simulink model "mainEMDmode"  (R2025b)
settings: Solver=VariableStepAuto  StartTime=0.0  StopTime=10  RelTol=1e-3
values from neighbouring files (symbols this model uses):
  B_m = (kfi^2*I_anl)/(V_an-R_a*I_anl)    (= 3.63928112965e-07)    [mainEMD.m]    (also in matlab.mat)
  Denominator = [L_a*J_m* + (L_a*B_m + J_m*R_a) + R_a*B_m+kfi^2]    [mainEMD.m]    (also in matlab.mat = 0.000519897304237)
  J_m = 1.16*10^-7    (= 1.16e-07)    [mainEMD.m]    (also in matlab.mat)
  kfi = 0.0225    [mainEMD.m]    (also in matlab.mat)
  L_a = 0.00137    [mainEMD.m]    (also in matlab.mat)
  Numerator = [kfi]    [mainEMD.m]    (also in matlab.mat = 0.0225)
  R_a = 37.5    [mainEMD.m]    (also in matlab.mat)
  T_n = 4.76*10^-3    (= 0.00476)    [mainEMD.m]    (also in matlab.mat)
  V_an = 24    [mainEMD.m]    (also in matlab.mat)
libraries: fl_lib x6, nesl_utility x5, ee_lib x2
settings Model: Creator=osakwe  LastModifiedBy=osakwe

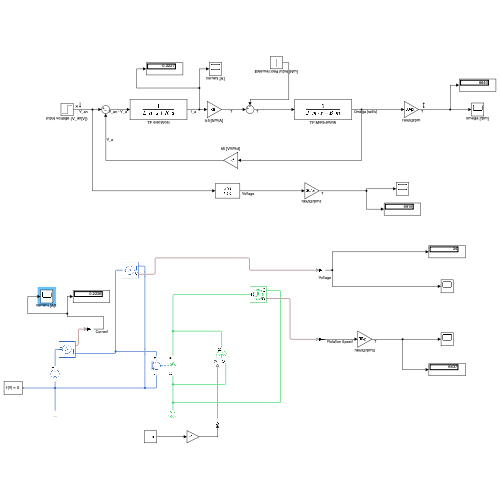
[thumbnail: Simulink's stored preview of the top-level diagram]
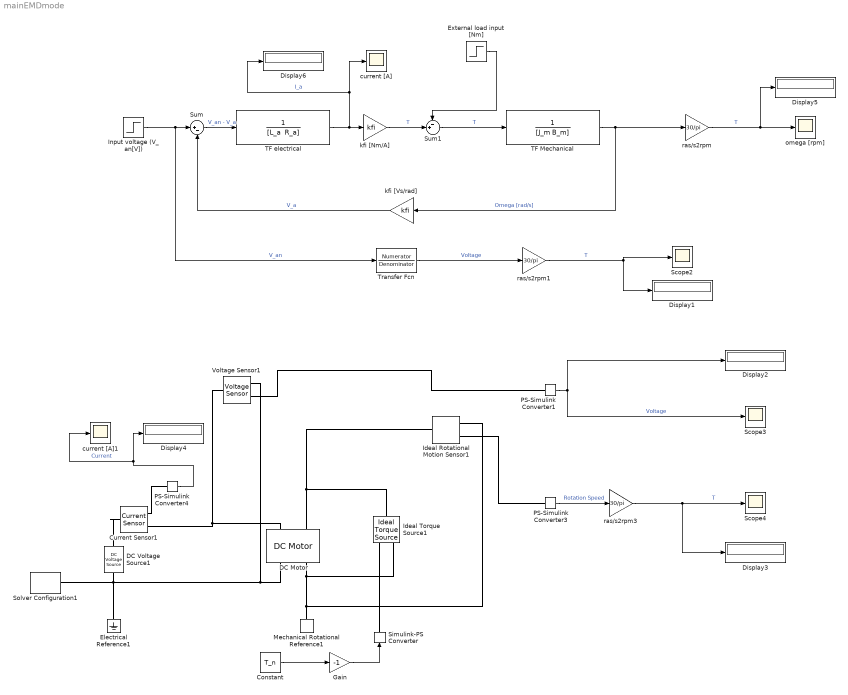
== system mainEMDmode ==
  Constant : Constant  Value=T_n
  Current Sensor1 : fl_lib/Electrical/Electrical Sensors/Current Sensor
  DC Motor : ee_lib/Electromechanical/Brushed Motors/DC Motor  field_option=ee.enum.field_option.pm  Rf=100 Ohm  Lf=1 H  Laf=0.15 H  If0=0 A  parameterization=ee.enum.dcparam_option.circuit_param  Ra=37.5 Ohm  La=1.37 mH  emf_or_torque=ee.enum.emf_or_torque.kv  Kv=0.00235849 V/rpm  Ki=6.876e-4 N*m/A  T_stall=14.4 mN*m  w_max=9920 rpm  w_rated=15000 rpm  P_rated=0.08 W  V_rated=1.5 V  lam_param=ee.enum.lam_param.damping  i_noload=16.8 mA  V_i_noload=1.5 V  J=1.16 cm^2*g  lam=B_m N*m*s/rad  speed0=0 rpm  alpha=3.93e-3 1/K  Tmeas=25 degC  thermal_mass=100 J/K  initial_temperature=25 degC
  DC Voltage Source1 : ee_lib/Additional Components/SPICE Sources/DC Voltage Source  DC=24 V
  Display{1..6} (6 alike) : Display
  Electrical Reference1 : fl_lib/Electrical/Electrical Elements/Electrical Reference
  External load input [Nm] : Step  Time=0  After=T_n  SampleTime=0
  Gain : Gain  Gain=-1
  Ideal Rotational Motion Sensor1 : fl_lib/Mechanical/Mechanical Sensors/Ideal Rotational Motion Sensor  reference=foundation.enum.MeasurementReference.difference  acceleration_port=false  velocity_port=true  position_port=false  wrap_angle=false  offset=0 rad
      settings: InternalSimscapePortConfiguration="{\"Bottom\":[],\"Left\":[{\"id\":\"R\",\"label\":\"R\",\"type\":\"foundation.mechanical.rotational.rotational\"}],\"Right\":[{\"id\":\"C\",\"label\":\"C\",\"type\":\"foundation.mechanical.rotational.rotational\"},{\"id\":\"W\",\"label\":\"W\",\"type\":\"output\"}],\"Top\":[]}"
  Ideal Torque Source1 : fl_lib/Mechanical/Mechanical Sources/Ideal Torque Source
  Input voltage (V_an[V]) : Step  Time=0  After=V_an  SampleTime=0
  Mechanical Rotational Reference1 : fl_lib/Mechanical/Rotational Elements/Mechanical Rotational Reference
  PS-Simulink Converter1 : nesl_utility/PS-Simulink Converter  PhysicalDomain=network_engine_domain  SubClassName=ps_output  LeftPortType=input  RightPortType=output  PseudoPeriodic=off  Frequencies=[]  VectorFormat=inherit  Unit=inherit  AffineConversion=off
  PS-Simulink Converter3 : nesl_utility/PS-Simulink Converter  PhysicalDomain=network_engine_domain  SubClassName=ps_output  LeftPortType=input  RightPortType=output  PseudoPeriodic=off  Frequencies=[]  VectorFormat=inherit  Unit=inherit  AffineConversion=off
  PS-Simulink Converter4 : nesl_utility/PS-Simulink Converter  PhysicalDomain=network_engine_domain  SubClassName=ps_output  LeftPortType=input  RightPortType=output  PseudoPeriodic=off  Frequencies=[]  VectorFormat=inherit  Unit=inherit  AffineConversion=off
  Scope2 : Scope
      settings: ActiveDisplayYMinimum=-1  ActiveDisplayYMaximum=1  DataLoggingVariableName=ScopeData2
  Scope3 : Scope
      settings: ActiveDisplayYMinimum=14  ActiveDisplayYMaximum=34  DataLoggingVariableName=ScopeData5
  Scope4 : Scope
      settings: Title=SIMSCAPE ANGULAR VELOCITY  ActiveDisplayYMinimum=-832.4286192839462  ActiveDisplayYMaximum=7466.9566783432829  YLabel=RPM  DataLoggingVariableName=ScopeData6
  Simulink-PS Converter : nesl_utility/Simulink-PS Converter  PhysicalDomain=network_engine_domain  SubClassName=ps_input  LeftPortType=input  RightPortType=output  PseudoPeriodic=off  Frequencies=[]  NoiseDistribution=none  NoiseParameters=[]  Unit=1  AffineConversion=off  FilteringAndDerivatives=provide  SimscapeFilterOrder=1  InputFilterTimeConstant=0.001  UdotUserProvided=0
  Solver Configuration1 : nesl_utility/Solver Configuration  PhysicalDomain=network_engine_domain  SubClassName=solver  LeftPortType=input  RightPortType=generic  Tones=[]  Harmonics=[]  SimulateNoise=off  Profile=off  UseLocalSampling=off  EnableSwitchedLinearOptims=on  FrequencyDomain=off  UseCCode=off  RelTol=0.001  AbsTol=0.001  MinStep=1e-09  ToWorkspace=off  RevertToSquareIcSolve=off  NumHomotopyIterations=100  PhasorMode=off  PhasorModeNumHarmonics=1  ConsistencySolver=NEWTON_XTOL_AFTER_FTOL  IndexReductionMethod=DerivativeReplacement  DoDC=off  ResidualTolerance=1e-09  ConsistencyTolSource=GLOBAL  ConsistencyAbsTol=0.001  ConsistencyRelTol=0.001  ConsistencyTolFactor=0.001  UseLocalSolver=off  LocalSolverChoice=NE_BACKWARD_EULER_ADVANCER  ResolveIndetEquations=on  FunctionEvalNumThread=1  LocalSolverSampleTime=0.001  DoFixedCost=off  MaxNonlinIter=3  MaxModeIter=2  ComputeImpulses=off  ImpulseIterations=2  LinearAlgebra=auto  LinearAlgebraNumThread=0  EquationFormulation=NE_TIME_EF  DelaysMemoryBudget=1024  AutomaticFiltering=on  FilteringTimeConstant=0.001  PartitionStorageMethod=AS_NEEDED  PartitionMemoryBudget=1024  PartitionMethod=ROBUST  MultibodyUseLocalSolver=off  MultibodyLocalSolverChoice=ODE1  MultibodyLocalSolverSampleTime=0.001
  Sum : Sum  Inputs=|+-
  Sum1 : Sum  Inputs=-+|
  TF Mechanical : TransferFcn  Denominator=[J_m B_m]
  TF electrical : TransferFcn  Denominator="[L_a  R_a]"
  Transfer Fcn : TransferFcn  Numerator=Numerator  Denominator=Denominator
  Voltage Sensor1 : fl_lib/Electrical/Electrical Sensors/Voltage Sensor
  current [A] : Scope
      settings: ActiveDisplayYMinimum=0.64117132473324245  ActiveDisplayYMaximum=0.643102729421688  DataLoggingVariableName=ScopeData3
  current [A]1 : Scope
      settings: ActiveDisplayYMinimum=-0.078481305185616052  ActiveDisplayYMaximum=0.70633198667053554
  kfi [Nm/A] : Gain  Gain=kfi
  kfi [Vs/rad] : Gain  Gain=kfi
  omega [rpm] : Scope
      settings: Title=BLOCK DIAGRAM ANGULAR VELOCITY  ActiveDisplayYMinimum=-832.80177547470191  ActiveDisplayYMaximum=7470.2676688358342  YLabel=RPM  DataLoggingVariableName=ScopeData4
  ras/s2rpm : Gain  Gain=30/pi
  ras/s2rpm1 : Gain  Gain=30/pi
  ras/s2rpm3 : Gain  Gain=30/pi
  wires:
  Sum/1 -> TF electrical/1  "V_an - V_a"
  Sum1/1 -> TF Mechanical/1  "T"
  ras/s2rpm/1 -> Display5/1, omega [rpm]/1  "T"
  TF electrical/1 -> Display6/1, current [A]/1, kfi [Nm/A]/1  "I_a"
  kfi [Vs/rad]/1 -> Sum/2  "V_a"
  Input voltage (V_an[V])/1 -> Transfer Fcn/1, Sum/1  "V_an"
  TF Mechanical/1 -> kfi [Vs/rad]/1, ras/s2rpm/1  "Omega [rad/s]"
  kfi [Nm/A]/1 -> Sum1/2  "T"
  External load input [Nm]/1 -> Sum1/1
  PS-Simulink Converter1/1 -> Display2/1, Scope3/1  "Voltage"
  PS-Simulink Converter4/1 -> current [A]1/1, Display4/1  "Current"
  Constant/1 -> Gain/1
  Gain/1 -> Simulink-PS Converter/1
  Transfer Fcn/1 -> ras/s2rpm1/1  "Voltage"
  ras/s2rpm1/1 -> Scope2/1, Display1/1  "T"
  PS-Simulink Converter3/1 -> ras/s2rpm3/1  "Rotation Speed"
  ras/s2rpm3/1 -> Display3/1, Scope4/1  "T"
  connections:
  Mechanical Rotational Reference1/LConn1 -- Ideal Rotational Motion Sensor1/RConn1 -- Ideal Torque Source1/RConn2 -- DC Motor/RConn2
  Ideal Rotational Motion Sensor1/LConn1 -- DC Motor/LConn2 -- Ideal Torque Source1/LConn1
  Voltage Sensor1/RConn2 -- Electrical Reference1/LConn1 -- Solver Configuration1/RConn1 -- DC Voltage Source1/RConn1 -- DC Motor/RConn1
  Ideal Rotational Motion Sensor1/RConn2 -- PS-Simulink Converter3/LConn1
  Voltage Sensor1/RConn1 -- PS-Simulink Converter1/LConn1
  Voltage Sensor1/LConn1 -- Current Sensor1/RConn2 -- DC Motor/LConn1
  Current Sensor1/LConn1 -- DC Voltage Source1/LConn1
  PS-Simulink Converter4/LConn1 -- Current Sensor1/RConn1
  Simulink-PS Converter/RConn1 -- Ideal Torque Source1/RConn1
